simulink model "ATOM_simple_planning_simulator"  (R2026a)
settings: Solver=ode4  StopTime=100  FixedStep=0.01
StopFcn:
  | % Put every new figure in the same MATLAB Figures window as a docked tab.
  | set(groot, 'defaultFigureWindowStyle', 'docked');
  | 
  | if exist('costmap_active', 'var') && ...
  |     exist('vehicle', 'var') && ...
  |     exist('parking_path', 'var') && ...
  |     ~isempty(parking_path)
  | 
  |      plotPlan(costmap_active, vehicle, parking_path);
  | 
  |  else
  | 
  |      warning('No valid parking path is available for plotting.');
  | 
  |  end
  | 
  |  PlotControllerReferences( ...
  |      out.controller_reference_log);
  | 
  |  PlotControllerTracking( ...
  |      out.controller_tracking_log);
  | 
model workspace (MAT data in the model file):
  vehicle : object (value not decoded)
symbols that are objects in the model workspace (value not decoded): vehicle
undefined symbols (not defined in the file): delta_f_LUT, gain4WS_LUT, k_ref_LUT, kappa_gain_BP, Ki, Kp, lateral, longitudinal, planning_validator, rr_gain_BP, rr_LUT, stanley, velocity_smoother
libraries: slpidlib x1
(part 7 of 8)

== matlab function ATOM_simple_planning_simulator/Subsystem2/parkingNMPC ==
  settings: updateMethod=DISCRETE  sampleTime=0.04
  data: tx input; path_length output; ty input; tqz input; tqw input; tdf input; tdr input; tvx input; tax input; max_q output; X input; Y input; s_now output; ey_now output; qz input; qw input; vx input; ax_meas input; df input; dr input; x_now output; veh input; longitudinal_mode output; df_rate_cmd output; dr_rate_cmd output; nmpc_info output; segment_done output; active_segment input; endpoint_error output; a_cmd_history input; costmap input; df_ref_out output; dr_ref_out output; t_ref input; s_ref input; x_ref input; y_ref input; psi_ref input; v_ref input; a_ref input; df_nom input; dr_nom input
function [path_length, max_q, s_now, ey_now, x_now, ...
    longitudinal_mode, df_rate_cmd, dr_rate_cmd, nmpc_info, ...
    segment_done, endpoint_error, ...
    df_ref_out, dr_ref_out] = parkingNMPC( ...
    tx,ty,tqz,tqw,tdf,tdr,tvx,tax, ...
    X,Y,qz,qw,vx,ax_meas,df,dr,veh, ...
    active_segment,a_cmd_history,costmap,t_ref,s_ref,x_ref,y_ref,psi_ref,v_ref,a_ref,df_nom,dr_nom)
%PARKINGNMPC  Steering NMPC of the ATOM parking chain, acados version (row 3).
%
%   Block    : ATOM_parking_chain/Subsystem2/parkingNMPC (MATLAB Function,
%              discrete, sample time Ts = 0.04 s, compiled to C).
%   Role     : computes the FRONT and REAR STEERING-RATE commands of the
%              4WS vehicle. Speed is NOT decided here: the separate block
%              parkingLongitudinalController (feed-forward + P law) computes
%              the acceleration; this block only predicts it.
%   Solver   : the optimal control problem is solved by acados through the
%              Simulink Function 'acadosSolve' (Subsystem2), which wraps
%              the generated S-function acados_solver_sfunction_atom_4ws_nmpc.
%              The OCP itself (model, cost, constraints, solver options) is
%              defined in MATLAB-Autoware/Acados/*.m and generated/compiled
%              by ATOM_Simulink_init.m.
%
%   WHAT HAPPENS EVERY 0.04 s
%     1  Supervisor: reference of the active gear segment, path progress
%        s_now, arrival / stop / wheel-alignment logic, longitudinal mode.
%     2  rolloutForAcados: predict 0.24 s through the steering dead time with
%        the 6 commands already queued (-> initial state x0bar of the OCP),
%        then 1.8 s more with the steering held (-> a_des profile, initial
%        guess, predicted path progress of every node).
%     3  acadosReferences: reference pose/steering of each OCP node, looked
%        up at the predicted path progress (path following).
%     4  buildCorridors: one obstacle-free rectangle per node from the
%        costmap (collision constraints of the OCP).
%     5  callAcados: pack everything into vectors and call acadosSolve
%        (skipped while the wheels are being aligned, status 7).
%     6  Status map: acados status -> controller status; unusable result ->
%        hold steering and stop.
%     7  Apply the FIRST command u0 only (receding horizon) and update the
%        internal copies of the commanded angle and of the delay queue.
%     8  Diagnostics nmpc_info (Scope2 ... Scope7).
%
%   TIMING
%     controller period Ts             0.04 s  (P.controlTs)
%     steering dead time (plant)       0.24 s  = nd = 6 controller steps
%     acceleration dead time (plant)   0.10 s  (handled inside predictStep)
%     OCP: N = 15 intervals of 0.12 s  -> 1.8 s, starting at t + 0.24 s
%
%   INPUTS (29)
%     tx,ty,tqz,tqw,tdf,tdr,tvx,tax  planner trajectory bus fields (x, y,
%                                    qz, qw, front/rear wheel angle, speed,
%                                    acceleration). NOT USED in this version;
%                                    kept so that the block wiring stays the
%                                    same. The reference comes from the
%                                    reference bus (t_ref ... dr_nom).
%     X, Y        [m]     rear-axle centre position (map frame)
%     qz, qw      [-]     yaw quaternion components (psi = 2*atan2(qz,qw))
%     vx          [m/s]   longitudinal speed (rear axle)
%     ax_meas     [m/s^2] longitudinal acceleration
%     df, dr      [rad]   measured front / rear wheel angles
%     veh         [-]     numeric vehicle-parameter vector (vehicleParameters.m)
%     active_segment      index of the gear segment being driven
%     a_cmd_history       3x1 acceleration commands already sent (oldest
%                         first), not yet through the 0.10 s dead time
%     costmap             occupancy-grid bus (info.resolution, width,
%                         height, origin; data int8 H x W: 0 free,
%                         100 occupied, -1 unknown)
%     t_ref, s_ref, x_ref, y_ref, psi_ref, v_ref, a_ref, df_nom, dr_nom
%                         reference of the active segment (time, arc
%                         length, pose, speed, acceleration, nominal
%                         front/rear steering), from the reference bus
%
%   OUTPUTS (13)
%     path_length        length of the active segment [m]       -> Display
%     max_q              max steering variation per metre        -> Display1
%     s_now              path progress [m]       -> longitudinal controller
%     ey_now             lateral error [m] (left +)              -> Scope1
%     x_now              current state [X;Y;psi;vx;df;dr;ax]     -> Display2
%     longitudinal_mode  0 follow plan, 1 slow creep, 2 stop -> long. ctrl
%     df_rate_cmd        front steering-rate command [rad/s]  -> df_cmd out
%     dr_rate_cmd        rear  steering-rate command [rad/s]  -> dr_cmd out
%                        (integrated to an angle by steeringRatetoAngle2,
%                        then delayed 0.24 s before the vehicle model)
%     nmpc_info          6x1 diagnostics (see the end of the main body)
%     segment_done       true when the segment end is reached, stopped and
%                        within the arrival tolerance -> next segment
%     endpoint_error     [distance to segment end [m]; heading error [deg]]
%     df_ref_out, dr_ref_out  reference steering at s_now [rad]
%
%   CONTROLLER STATUS (nmpc_info(6), Scope7)
%     0 acados converged within 0.04 s     1 usable (slow or acados 2)
%     2 unusable -> hold steering, stop    3 baseline mode (use_nmpc false)
%     4 segment done, outside 0.05 m / 2 deg   5 stopped at the end but
%       outside the arrival tolerance 0.20 m / 5 deg
%     7 wheel alignment (vehicle held)     8 cusp hand-off (see note there)
%
%   EXTERNAL DEPENDENCIES
%     acadosSolve     Simulink Function in Subsystem2 (scoped)
%     bicycleGetPose  MATLAB-Autoware/Functions (used by predictStep)

% ---------------------------------------------------------------------
% Persistent state (kept between calls, reset only at simulation start)
%   ref                       reference structure of the active segment
%   s_prev                    path progress of the previous call [m]
%   buf                       6x2 steering-angle commands already sent and
%                             still inside the 0.24 s dead time [front rear],
%                             oldest first
%   terminal_creep_steps      leftover of an earlier version: set but never
%                             read (cleanup candidate)
%   previous_active_segment   to detect a segment change
%   steering_command_state    last commanded angles [front rear] = output
%                             of the external rate-to-angle integrator
%   steering_alignment_pending  true until the wheels reach the start
%                             angles of the new segment
% ---------------------------------------------------------------------
persistent ref s_prev buf terminal_creep_steps
persistent previous_active_segment
persistent steering_command_state
persistent steering_alignment_pending
persistent solver_failure_count

N  = 15;   % OCP intervals; here only the size of U_selected (row 1 is used)
nd = 6;    % steering dead time in controller steps: 0.24 s / 0.04 s

% ===================== 1. SEGMENT BOOKKEEPING =========================
% Detect a change of the active gear segment (forward <-> reverse).
if isempty(previous_active_segment)
    previous_active_segment = active_segment;
    segment_changed = false;
else
    segment_changed = ...
        active_segment ~= previous_active_segment;

    previous_active_segment = active_segment;
end

% Build the reference during the first execution.
if isempty(ref)
    ref = buildRef( ...
        t_ref,s_ref,x_ref,y_ref,psi_ref,v_ref,a_ref, ...
        df_nom,dr_nom);
end

if isempty(s_prev)
    s_prev = 0;
end

if isempty(buf)
    % Initialize the delayed-command history from the measured wheel angles
    % (at start-up nothing different has been commanded yet).
    buf = repmat([df, dr], nd, 1);
end

if isempty(steering_command_state)
    % The commanded angles start equal to the measured wheel angles.
    steering_command_state = [df,dr];
end

% History of acceleration commands already sent to the vehicle.
% Three samples are retained because the acceleration delay is 0.10 s,
% equivalent to 2.5 controller intervals at Ts = 0.04 s.
% Acceleration commands sampled externally every 0.04 seconds.
aBuf = a_cmd_history;

if isempty(terminal_creep_steps)
    terminal_creep_steps = 0.0;
end

if isempty(solver_failure_count)
    solver_failure_count = 0;
end

if isempty(steering_alignment_pending)
    % The first segment also starts with a wheel-alignment check.
    steering_alignment_pending = true;
end

% Rebuild the reference once when the segment changes; restart the path
% progress and request a wheel alignment for the new segment.
if logical(segment_changed)
    ref = buildRef( ...
        t_ref,s_ref,x_ref,y_ref,psi_ref,v_ref,a_ref, ...
        df_nom,dr_nom);
    s_prev = 0;
    terminal_creep_steps = 0.0;
    steering_alignment_pending = true;
end

% ===================== 2. WHERE IS THE CAR ON THE PATH ================
path_length = ref.s(end); max_q = max(ref.q);
[s_new, ey_now] = whereOnPath(ref, X, Y, s_prev);
s_now  = min(max(s_new, s_prev), s_prev + 0.5);   % never backwards, never a big jump forward

% Reference steering at the current progress (outputs for logging).
df_ref_out = lookupS(ref.s, ref.df, s_now);
dr_ref_out = lookupS(ref.s, ref.dr, s_now);

s_prev = s_now;

% --- the state of the car right now ---
psi   = 2*atan2(qz, qw);                              % yaw from the quaternion
x_now = [X; Y; psi; vx; df; dr; ax_meas];             % 7-state vector of the internal prediction model
P     = carNumbers(veh);                              % vehicle, actuator and footprint numbers
M = mapNumbers(costmap);                              % costmap as doubles (0..1, <0 unknown)

% Collision measure of the CURRENT pose (monitor only, Scope2):
% < 0 free, > 0 the expanded footprint overlaps an obstacle cell.
current_collision_constraint = ...
    poseCollisionConstraint(X,Y,psi,P,M);

% Remaining path distance used by the maneuver supervisor.
d_left = max(ref.s(end) - s_now, 0);

% The segment is complete only after reaching its end and stopping.
% Actual distance from the vehicle's rear axle to the segment endpoint.
endpoint_distance = hypot( ...
    X - ref.X(end), ...
    Y - ref.Y(end));

% Heading error relative to the segment endpoint, wrapped to [-pi, pi].
heading_difference = psi - ref.psi(end);

endpoint_heading_error = atan2( ...
    sin(heading_difference), ...
    cos(heading_difference));

% ===================== 3. ARRIVAL, STOP AND ALIGNMENT SUPERVISION =====
%
% Precise tolerance:
% Used to evaluate the final tracking quality.
%
% Arrival tolerance:
% Used to decide whether the stopped vehicle may proceed to the next
% forward/reverse segment.

end_distance_tolerance = 0.05;       % [m]
end_heading_tolerance  = 2*pi/180;   % [rad]

arrive_distance_tolerance = 0.20;    % [m]
arrive_heading_tolerance = 5*pi/180; % [rad]

stop_speed_tolerance = 0.02;         % [m/s]

% Because s_now is not allowed to decrease, end_reached remains true
% after the vehicle reaches the final path progress.
end_reached = ...
    d_left <= 0.02;

% High-accuracy endpoint condition.
pose_acceptable = ...
    (endpoint_distance <= end_distance_tolerance) && ...
    (abs(endpoint_heading_error) <= end_heading_tolerance);

% Practical condition for authorizing the next gear segment.
pose_arrived = ...
    (endpoint_distance <= arrive_distance_tolerance) && ...
    (abs(endpoint_heading_error) <= arrive_heading_tolerance);

% The vehicle must be nearly stationary before changing segments.
stopped = ...
    abs(vx) <= stop_speed_tolerance;

% Steering must be positioned for the new segment before motion begins.
steering_alignment_tolerance = 2*pi/180;

segment_start_front_steering = ref.df(1);
segment_start_rear_steering  = ref.dr(1);

front_steering_aligned = ...
    abs(df-segment_start_front_steering) <= ...
    steering_alignment_tolerance;

rear_steering_aligned = ...
    abs(dr-segment_start_rear_steering) <= ...
    steering_alignment_tolerance;

steering_aligned = ...
    front_steering_aligned && ...
    rear_steering_aligned;

% Release the alignment hold only after the measured wheels - not merely
% the requested commands - have reached the new segment's starting angles.
if steering_alignment_pending && stopped && steering_aligned
    steering_alignment_pending = false;
end

steering_alignment_active = steering_alignment_pending;

% Advance to the next segment only after reaching the endpoint progress,
% stopping, and satisfying the practical arrival tolerance.
segment_done = ...
    end_reached && ...
    stopped && ...
    pose_arrived;

% If the vehicle stops outside the arrival tolerance, keep the current
% segment active and report the failure through the controller status.
arrival_failed = ...
    end_reached && ...
    stopped && ...
    ~pose_arrived;

% Permanent endpoint diagnostics:
%   element 1: position error [m]
%   element 2: signed heading error [deg]
endpoint_error = [ ...
    endpoint_distance; ...
    endpoint_heading_error*180/pi];

% Longitudinal modes (read by parkingLongitudinalController):
%   0 = follow the planned velocity profile
%   1 = slow terminal approach
%   2 = stop
longitudinal_mode = 0.0;

if steering_alignment_active

    % Keep the vehicle stopped while the wheels align.
    longitudinal_mode = 2.0;

elseif end_reached

    if pose_arrived
        % Correct endpoint pose reached.
        longitudinal_mode = 2.0;
    else
        % Continue slowly to correct the endpoint pose.
        % S1: creep only while the endpoint is still ahead in the driving
        % direction, and for at most max_creep_steps samples
        % (150 x 0.04 s = 6 s, i.e. 0.30 m at 0.05 m/s). Otherwise stop;
        % once stopped, arrival_failed reports controller status 5.
        max_creep_steps = 150;
        endpoint_ahead = ref.gear*( ...
            cos(psi)*(ref.X(end) - X) + sin(psi)*(ref.Y(end) - Y));
        if endpoint_ahead <= 0.02
            % Endpoint beside or behind the car: creeping cannot reach it.
            terminal_creep_steps = max_creep_steps;
        end
        if terminal_creep_steps < max_creep_steps
            terminal_creep_steps = terminal_creep_steps + 1;
            longitudinal_mode = 1.0;
        else
            % Creep abandoned: stop (latched until the segment changes).
            longitudinal_mode = 2.0;
        end
    end

end

% ===================== 4. STEERING: acados NMPC =======================
use_nmpc = true;      % false = D1 baseline (follow the plan blindly)

if use_nmpc

    % Collision tolerance of the cusp hand-off check (section 4.6).
    collision_tolerance = 1e-6;

    % ---- 4.1 Prediction that prepares the OCP -----------------------
    % Phase 1: 0.24 s with the 6 queued commands -> x0bar (OCP state at
    % t + 0.24 s). Phase 2: 15 x 0.12 s with the steering held ->
    % aDes (acceleration entering the lag, per interval), xGuess
    % (initial guess) and sNode (predicted path progress of each node).
    [x0bar, aDes, xGuess, sNode] = rolloutForAcados( ...
        x_now, aBuf, buf, steering_command_state, ...
        s_now, ref, P, longitudinal_mode);

    % ---- 4.2 References at the predicted path progress of each node --
    acados_reference = acadosReferences(ref, sNode);

    % ---- 4.3 Obstacle corridor for every node, from the costmap -------
    [Acorr, bcorr] = buildCorridors(x0bar, acados_reference, P, M);

    % ---- 4.4 Solve with acados ----------------------------------------
    % Skipped while the supervisor aligns the wheels (status 7): the
    % steering command is overridden by the alignment logic anyway.
    if steering_alignment_active
        u0_acados       = zeros(2,1);
        acados_status   = 0;
        acados_sqp_iter = 0;
        solve_time      = 0;
    else
        [u0_acados, ~, acados_status, acados_sqp_iter, solve_time] = ...
            callAcados(x0bar, acados_reference, aDes, xGuess, Acorr, bcorr);
    end

    % ---- 4.5 Check the returned first command and map the status ------
    acados_rate_bound = 1.0;    % must equal atomCfg.omegaMax (compiled in the solver)
    finite_solution = all(isfinite(u0_acados));
    inside_bounds   = all(abs(u0_acados) <= acados_rate_bound + 1e-6);

    % Translate the acados status into the controller status.
    %   acados 0           -> 0 (1 if slower than the 0.04 s period)
    %   acados 2 (max it.) -> 1 (usable, not fully converged)
    %   anything else      -> 2 (unusable)
    if acados_status == 0 && finite_solution && inside_bounds
        if solve_time > P.controlTs
            controller_status = 1;
        else
            controller_status = 0;
        end
    elseif acados_status == 2 && finite_solution && inside_bounds
        controller_status = 1;
    else
        controller_status = 2;
    end

    % Endpoint-arrival diagnostics (same as the fmincon version).
    % S3: a non-converged solve (acados status ~= 0) is accepted only
    % for a short time. After more than max_solver_failures consecutive
    % failures (5 x 0.04 s = 0.2 s) the command is treated as unusable:
    % controller status 2 -> hold the steering and stop. The stop is
    % latched: once triggered, the counter is no longer reset.
    max_solver_failures = 5;
    if solver_failure_count <= max_solver_failures
        if acados_status ~= 0
            solver_failure_count = solver_failure_count + 1;
        else
            solver_failure_count = 0;
        end
    end
    if solver_failure_count > max_solver_failures
        controller_status = 2;
    end

    % Endpoint-arrival diagnostics (same as the fmincon version).
    if controller_status ~= 2
        if arrival_failed
            controller_status = 5;
        elseif segment_done && ~pose_acceptable
            controller_status = 4;
        end
    end

    % Steering-rate plan used by the rest of the function. Only the FIRST
    % row is applied (receding horizon); the other rows stay zero.
    % Status 2: rate 0 = hold the last issued steering command.
    U_selected = zeros(N,2);
    if controller_status ~= 2
        U_selected(1,1:2) = u0_acados(:).';
    else
        % No valid (collision-free) steering plan: hold steering and stop.
        longitudinal_mode = 2.0;
    end

    % ---- Wheel alignment at a gear change (status 7) ------------------
    % Align the wheels directly while the vehicle is stopped. This does not
    % move the vehicle body. While steering alignment is pending, keep the
    % vehicle stopped and do not allow the NMPC solution to compete with it.
    if steering_alignment_active

        longitudinal_mode = 2.0;
        controller_status = 7;

        % Zero rate holds the current desired steering angles while the
        % vehicle is still coming to rest.
        U_selected = zeros(N,2);

        % Begin changing the steering only after the vehicle has stopped:
        % rate that reaches the start angles in one step, limited to the
        % actuator rate limit P.rateLim (5 rad/s).
        if stopped

            target_front_angle = max( ...
                -P.steerMax, ...
                min(P.steerMax,segment_start_front_steering));

            target_rear_angle = max( ...
                -P.steerMax, ...
                min(P.steerMax,segment_start_rear_steering));

            alignment_front_rate = ...
                (target_front_angle-steering_command_state(1))/P.controlTs;

            alignment_rear_rate = ...
                (target_rear_angle-steering_command_state(2))/P.controlTs;

            alignment_front_rate = max( ...
                -P.rateLim, ...
                min(P.rateLim,alignment_front_rate));

            alignment_rear_rate = max( ...
                -P.rateLim, ...
                min(P.rateLim,alignment_rear_rate));

            U_selected(1,1:2) = ...
                [alignment_front_rate,alignment_rear_rate];
        end
    end

    % ---- Outputs: the two steering-rate commands -----------------------
    selected_input = U_selected(1,:);

    df_rate_cmd = selected_input(1);
    dr_rate_cmd = selected_input(2);

    selected_rate = selected_input(1:2);

    % Mirror the external rate-to-angle integrator (steeringRatetoAngle2)
    % inside the NMPC: commanded angle after this step.
    sent_angle_trajectory = expandSteeringRatePlan( ...
        selected_rate,steering_command_state,P);

    steering_command_state = ...
        sent_angle_trajectory(end,:);

    % Push the new command into the 0.24 s delay queue (keep the last 6).
    updated_delay_history = ...
        [buf;sent_angle_trajectory];

    buf = updated_delay_history(end-nd+1:end,:);

    % Status 7 means the vehicle is intentionally stationary while its
    % measured steering aligns with the new segment.
    if steering_alignment_active && ...
            (controller_status == 0 || controller_status == 1)

        controller_status = 7;
    end

    % ---- 4.6 Cusp hand-off (status 8) ---------------------------------
    % Terminal creep is collision-infeasible, but the stopped vehicle is
    % currently collision-free and sufficiently close to the cusp.
    % Authorize the gear change so the next segment can move away from
    % the obstacle instead of repeating an impossible creep forever.
    % NOTE: this needs controller_status == 6, which only the fmincon
    % version produced. In this acados version it can never trigger.

    cusp_recovery_distance_tolerance = 0.25;        % [m]
    cusp_recovery_heading_tolerance  = 10*pi/180;   % [rad]

    safe_cusp_handoff = ...
        (controller_status == 6) && ...
        arrival_failed && ...
        ~steering_alignment_active && ...
        (current_collision_constraint <= collision_tolerance) && ...
        (endpoint_distance <= cusp_recovery_distance_tolerance) && ...
        (abs(endpoint_heading_error) <= ...
        cusp_recovery_heading_tolerance);

    if safe_cusp_handoff
        segment_done = true;
        controller_status = 8;
    end

    % ---- 4.7 Diagnostics (Demux -> Scope2 ... Scope7) -----------------
    %   1 collision monitor of the CURRENT pose (> 0 = overlaps an obstacle)
    %   2 acados status (0 converged, 2 max iterations, 4 QP failure, ...)
    %   3 acados CPU time [s]
    %   4 SQP iterations
    %   5 acceleration entering the lag at node 0 (a_des) [m/s^2]
    %   6 controller status
    nmpc_info = [ ...
        double(current_collision_constraint); ...
        double(acados_status); ...
        double(solve_time); ...
        double(acados_sqp_iter); ...
        double(aDes(1)); ...
        double(controller_status)];
else
    % ===================== BASELINE (use_nmpc = false) ===================
    % Follow the planned steering angles at the current progress, without
    % optimisation (comparison mode only).
    target_front_angle = lookupS(ref.s,ref.df,s_now);
    target_rear_angle  = lookupS(ref.s,ref.dr,s_now);

    % Convert the required angle changes into steering-rate commands.
    df_rate_cmd = ...
        (target_front_angle-steering_command_state(1))/P.controlTs;

    dr_rate_cmd = ...
        (target_rear_angle-steering_command_state(2))/P.controlTs;

    % Apply the actuator steering-rate limit.
    df_rate_cmd = max(-P.rateLim,min(P.rateLim,df_rate_cmd));
    dr_rate_cmd = max(-P.rateLim,min(P.rateLim,dr_rate_cmd));

    % Mirror the steering command actually selected in baseline mode.
    selected_rate = [df_rate_cmd,dr_rate_cmd];

    sent_angle_trajectory = expandSteeringRatePlan( ...
        selected_rate,steering_command_state,P);

    steering_command_state = sent_angle_trajectory(end,:);

    updated_delay_history = [buf;sent_angle_trajectory];
    buf = updated_delay_history(end-nd+1:end,:);

    nmpc_info = [0; 0; 0; 0; 0; 3];
end
end

%==========================================================================
%  GENERAL HELPERS (vehicle numbers, costmap, prediction model, path)
%==========================================================================

%--------------------------------------------------------------------------
function P = carNumbers(veh)
%CARNUMBERS  Vehicle, actuator, timing and footprint numbers in one struct.
%   veh is the numeric vector of vehicleParameters.m:
%     veh(3) wheel base, veh(4) track, veh(5)/veh(6) front/rear overhang,
%     veh(7)/veh(8) left/right overhang, veh(10) max wheel angle,
%     veh(15) velocity limit, veh(16) acceleration limit,
%     veh(18) actuator steering-rate limit, veh(19) acceleration dead time,
%     veh(20) acceleration time constant, veh(22) steering time constant.
%   All fields must be created before the structure is read (code generation).

collisionMargin = 0.4;%0.5;     % total margin around the car [m] (0.25 m per face)

% Controller and internal prediction timing.
controlTs    = 0.04;
predictionTs = 0.04;

P.L        = veh(3);       % wheel base 2.0 m
P.steerMax = veh(10);      % max wheel / command angle 0.70 rad
P.aMax     = veh(16);      % acceleration clip in the prediction 7.0 m/s^2
P.rateLim  = veh(18);      % actuator steering-rate limit 5 rad/s
P.tau      = veh(22);      % steering time constant 0.27 s

% Speed clip of the prediction. veh(15) is the simulator velocity limit
% (50 m/s), so in practice this clip is never active.
P.vMax = veh(15);       % Prediction clip
P.vStateMax = veh(15);  % leftover of the fmincon speed constraint: not used any more

P.controlTs = controlTs;
P.predictionTs = predictionTs;
P.substepsPerControl = round( ...
    controlTs/predictionTs);   % = 1: one prediction step per command

P.accDelay = veh(19);      % 0.10 s; not used: the delay is built into predictStep / aBuf
P.accTau   = veh(20);      % acceleration time constant 0.10 s
P.aCmdMax  = 1.0; % Match a_cmd_limit in parkingLongitudinalController.

% Expanded footprint in vehicle coordinates (origin = rear-axle centre,
% l forward, w to the left): l in [footprintBack, footprintFront],
% w in [-footprintHalfWidth, +footprintHalfWidth].
P.footprintMargin = collisionMargin;     % not used elsewhere

P.footprintBack = ...
    -(veh(6) + collisionMargin/2);         % -0.71 m

P.footprintFront = ...
    veh(3) + veh(5) + collisionMargin/2;   % +2.71 m

P.footprintHalfWidth = ...
    (veh(4) + veh(7) + veh(8) + collisionMargin)/2;   % 1.328 m
end

%--------------------------------------------------------------------------
function M = mapNumbers(costmap)
%MAPNUMBERS  Costmap bus -> doubles used by the collision code.
%   Cell (ix, iy), zero-based, is a square of side res centred at
%   (originX + ix*res, originY + iy*res). grid = data/100:
%   0 free, 1 occupied, -0.01 unknown (unknown is treated as an obstacle).

resolution = double(costmap.info.resolution);

M.res = resolution;
M.width = double(costmap.info.width);
M.height = double(costmap.info.height);

M.originX = double(costmap.info.origin.position.x);
M.originY = double(costmap.info.origin.position.y);

M.grid = double(costmap.data)/100;

M.cellHalf = resolution/2;
end

%--------------------------------------------------------------------------
function [x1,aBuf1,df_raw,dr_raw,vx_raw] = predictStep( ...
    x0,aBuf,aCmd,dfc,drc,P)
%PREDICTSTEP  Discrete vehicle model over one 0.04 s controller interval.
%   x0   = [X; Y; psi; vx; df; dr; ax]   state at the start of the step
%   aBuf = acceleration commands inside the 0.10 s dead time (oldest first)
%   aCmd = acceleration command issued in this step (enters aBuf)
%   dfc, drc = steering-angle commands reaching the actuator in this step
%   x1   = state after 0.04 s;  aBuf1 = updated acceleration queue.
%   df_raw, dr_raw, vx_raw are the unclipped values (were used by the
%   fmincon constraints; the acados roll-out does not use them).
%   This is the model used to compute x0bar, a_des and the initial guess.

X   = x0(1);
Y   = x0(2);
psi = x0(3);
vx  = x0(4);
df  = x0(5);
dr  = x0(6);
ax  = x0(7);

%% Steering actuator: first-order lag (tau = 0.27 s) with rate limit
ddf = max( ...
    -P.rateLim, ...
    min(P.rateLim,(dfc-df)/P.tau));

ddr = max( ...
    -P.rateLim, ...
    min(P.rateLim,(drc-dr)/P.tau));

df_raw = df + P.predictionTs*ddf;
dr_raw = dr + P.predictionTs*ddr;

df1 = max(-P.steerMax,min(P.steerMax,df_raw));
dr1 = max(-P.steerMax,min(P.steerMax,dr_raw));

%% Acceleration delay and actuator lag

% The 0.04 s interval is divided into two 0.02 s parts.
h = 0.5*P.predictionTs;

% For a 0.10 s transport delay, the delayed command changes halfway
% through the current 0.04 s interval.
aDelayedFirst  = aBuf(1);
aDelayedSecond = aBuf(2);

% First half of the acceleration-actuator response.
axHalf = ax + ...
    h*(aDelayedFirst-ax)/P.accTau;

axHalf = max( ...
    -P.aMax, ...
    min(P.aMax,axHalf));

% Second half of the acceleration-actuator response.
ax1 = axHalf + ...
    h*(aDelayedSecond-axHalf)/P.accTau;

ax1 = max( ...
    -P.aMax, ...
    min(P.aMax,ax1));

% Integrate longitudinal acceleration over the two half-steps (trapezoid).
deltaVFirst = ...
    0.5*h*(ax+axHalf);

deltaVSecond = ...
    0.5*h*(axHalf+ax1);

vxFromAcceleration = ...
    vx + deltaVFirst + deltaVSecond;

% Steering changes during this controller interval, so use its
% midpoint value when predicting the vehicle motion.
dfMid = 0.5*(df+df1);
drMid = 0.5*(dr+dr1);

% Match the longitudinal-velocity equation used by Vehicle_Model:
% dvx/dt = a + yawRate * v * sin(dr), with v = vx / cos(dr).
vxMidForCoupling = ...
    0.5*(vx+vxFromAcceleration);

vehicleSpeedMid = ...
    vxMidForCoupling/max(cos(drMid),0.1);

yawRateMid = ...
    (vxMidForCoupling/P.L) * ...
    (tan(dfMid)-tan(drMid));

rearSteeringVelocityTerm = ...
    yawRateMid*vehicleSpeedMid*sin(drMid);

% Unclipped prediction (returned as vx_raw).
vx_raw = vxFromAcceleration + ...
    P.predictionTs*rearSteeringVelocityTerm;

% Keep the numerical guard for state propagation.
vx1 = max(-P.vMax,min(P.vMax,vx_raw));

% Store the acceleration command predicted for the current cycle.
aBuf1 = [aBuf(2:end); aCmd];

%% Vehicle motion: arc of the rear-axle point (bicycleGetPose)

vxMid = 0.5*(vx+vx1);

dRear = ...
    vxMid*P.predictionTs/max(cos(drMid),0.1);   % distance travelled by the rear-axle point

[X1,Y1,psi1] = bicycleGetPose( ...
    X,Y,psi,dfMid,drMid,P.L,dRear);


x1 = [X1;Y1;psi1;vx1;df1;dr1;ax1];


end

%-------------------------------------------------------------------------
function angle_commands = expandSteeringRatePlan( ...
    rate_commands,initial_angle_command,P)
%EXPANDSTEERINGRATEPLAN  Integrate steering-rate commands into angles.
%   Same law as the external block steeringRatetoAngle2:
%     c(k+1) = sat( c(k) + 0.04 * sat(rate, +-P.rateLim), +-P.steerMax )
%   rate_commands: n x 2 [front rear] rates; initial_angle_command: 1 x 2.
%   angle_commands: (n*substeps) x 2 commanded angles after each sub-step.
%   Called with one row (the command applied now): the result updates
%   steering_command_state and the delay queue buf.

number_of_rate_commands = size(rate_commands,1);
substeps_per_command = P.substepsPerControl;

number_of_angle_samples = ...
    number_of_rate_commands*substeps_per_command;

angle_commands = zeros(number_of_angle_samples,2);

front_command = initial_angle_command(1);
rear_command  = initial_angle_command(2);

sample_index = 0;

for k = 1:number_of_rate_commands

    front_rate = max( ...
        -P.rateLim, ...
        min(P.rateLim,rate_commands(k,1)));

    rear_rate = max( ...
        -P.rateLim, ...
        min(P.rateLim,rate_commands(k,2)));

    for j = 1:substeps_per_command

        front_command = max( ...
            -P.steerMax, ...
            min(P.steerMax, ...
            front_command + ...
            P.predictionTs*front_rate));

        rear_command = max( ...
            -P.steerMax, ...
            min(P.steerMax, ...
            rear_command + ...
            P.predictionTs*rear_rate));

        sample_index = sample_index + 1;

        angle_commands(sample_index,1) = front_command;
        angle_commands(sample_index,2) = rear_command;
    end
end
end

%--------------------------------------------------------------------------
function a_cmd = longitudinalCommandPrediction( ...
    ref, s, vx, longitudinal_mode, P)
%LONGITUDINALCOMMANDPREDICTION  Copy of the law of parkingLongitudinalController.
%   Predicts the acceleration command the separate longitudinal controller
%   will issue at progress s and speed vx:
%     a_cmd = sat( a_ff + Kp*(v_ref - vx), +-P.aCmdMax )
%   mode 0: plan (v_ref, a_ref at s, Kp = 1); mode 1: creep at 0.05 m/s in
%   the segment gear; mode 2: stop (v_ref = 0, Kp_stop = 5).
%   Braking feed-forward is dropped while the car is already slower than
%   its reference in the gear direction.

Kp = 1.0;
Kp_stop = 5.0;
terminal_creep_speed = 0.05;

v_ref = lookupS(ref.s,ref.v,s);
a_ref = lookupS(ref.s,ref.a,s);

gear = ref.gear;             % +1 forward, -1 reverse
Kp_active = Kp;

if longitudinal_mode == 2.0

    % Stop mode.
    v_ref = 0.0;
    a_ref = 0.0;
    Kp_active = Kp_stop;

elseif longitudinal_mode == 1.0

    % Terminal-creep mode.
    v_ref = gear*terminal_creep_speed;
    a_ref = 0.0;

end

speed_error = v_ref-vx;

speed_in_gear = gear*vx;
reference_speed_in_gear = gear*v_ref;
feedforward_in_gear = gear*a_ref;

a_feedforward = a_ref;

% Apply braking feedforward only while the vehicle is moving faster
% than its reference in the intended gear direction.
if feedforward_in_gear < 0.0 && ...
        speed_in_gear <= reference_speed_in_gear

    a_feedforward = 0.0;

end

a_unsaturated = ...
    a_feedforward + Kp_active*speed_error;

a_cmd = max( ...
    -P.aCmdMax, ...
    min(P.aCmdMax,a_unsaturated));

end

%--------------------------------------------------------------------------
function v = lookupS(sv, vv, s)
%LOOKUPS  Linear interpolation of vv(sv) at s, held constant outside the range.
%   Used for every reference lookup by arc length (or by time).
n = numel(sv);
v = vv(n);
if s <= sv(1), v = vv(1); return; end
if s >= sv(n), return; end
for i = 1:n-1
    if s <= sv(i+1)
        ds = sv(i+1) - sv(i);
        if ds < 1e-12
            v = vv(i+1);
        else
            v = vv(i) + (s - sv(i))/ds*(vv(i+1) - vv(i));
        end
        return;
    end
end
end

%--------------------------------------------------------------------------
function ref = buildRef( ...
    t_ref,s_ref,x_ref,y_ref,psi_ref,v_ref,a_ref, ...
    df_nom,dr_nom)
%BUILDREF  Reference structure of the active segment.
%   Fields: t, s, X, Y, psi, v, a, df, dr (column vectors), q = steering
%   variation per metre (max over front/rear), gear = sign of the first
%   non-zero reference speed (+1 forward, -1 reverse).

% Local arrays
t   = t_ref(:);
s   = s_ref(:);
Xr  = x_ref(:);
Yr  = y_ref(:);
psir = psi_ref(:);
vr  = v_ref(:);
ar  = a_ref(:);
dfr = df_nom(:);
drr = dr_nom(:);

n = numel(t);

%% Steering variation per metre

q = zeros(n,1);

for i = 1:n-1

    ds = max(s(i+1)-s(i),1e-9);

    q(i) = max( ...
        abs(dfr(i+1)-dfr(i)), ...
        abs(drr(i+1)-drr(i))) / ds;

end

if n > 1
    q(n) = q(n-1);
else
    q(1) = 0.0;
end

%% Forward or reverse gear

gear = 1;

for i = 1:n

    if abs(vr(i)) > 1e-6
        gear = sign(vr(i));
        break;
    end

end

%% Create every structure field after calculations are complete

ref.t    = t;
ref.s    = s;
ref.X    = Xr;
ref.Y    = Yr;
ref.psi  = psir;
ref.v    = vr;
ref.a    = ar;
ref.df   = dfr;
ref.dr   = drr;
ref.q    = q;
ref.gear = gear;

end

%--------------------------------------------------------------------------
function [s, ey] = whereOnPath(ref, X, Y, s_guess)
%WHEREONPATH  Closest point on the route to (X,Y).
%   s  : how far along the route that point is [m]
%   ey : how far to the side the car is (left positive) [m]
%   First searches the segments within 1.5 m of s_guess; if none is found,
%   searches the whole route.
n = numel(ref.s);
best = inf;  s = s_guess;  ey = 0;
win  = 1.5;

for pass = 1:2
    for i = 1:n-1
        if abs(ref.s(i) - s_guess) > win
            continue;
        end
        ax = ref.X(i);   ay = ref.Y(i);
        bx = ref.X(i+1); by = ref.Y(i+1);
        L2 = (bx-ax)^2 + (by-ay)^2;
        t  = ((X-ax)*(bx-ax) + (Y-ay)*(by-ay)) / max(L2, 1e-12);
        t  = min(max(t, 0), 1);
        px = ax + t*(bx-ax);   py = ay + t*(by-ay);
        d2 = (X-px)^2 + (Y-py)^2;
        if d2 < best
            best = d2;
            s  = ref.s(i) + t*(ref.s(i+1) - ref.s(i));
            ey = sign((bx-ax)*(Y-ay) - (by-ay)*(X-ax)) * sqrt(d2);
        end
    end
    if best < inf, break; end
    win = inf;
end
end

%--------------------------------------------------------------------------
function cPose = poseCollisionConstraint(X,Y,psi,P,M)
%POSECOLLISIONCONSTRAINT  Collision measure of ONE vehicle pose (SAT test).
%   In this version it is only a MONITOR of the current pose (Scope2 and the
%   cusp check); the OCP uses the corridors of buildCorridors instead.
%     cPose < 0 : collision-free (about minus the clearance, >= -1 m)
%     cPose = 0 : touching an obstacle cell or the map boundary
%     cPose > 0 : the expanded footprint overlaps an obstacle / leaves the map
%   Separating-axis test between the expanded footprint rectangle and every
%   occupied or unknown cell near the car (world axes and vehicle axes).

% Nearby obstacles begin influencing the constraint from this distance.
% This is not an additional vehicle safety margin.
influenceDistance = 1.0;

% Prevent exact geometric touching from being accepted because of
% numerical round-off.
numericalClearance = 1e-4;

ct = cos(psi);
st = sin(psi);

%% Enlarged vehicle rectangle

back = P.footprintBack;
front = P.footprintFront;
halfWidth = P.footprintHalfWidth;

vehicleCentreOffset = 0.5*(front + back);
vehicleHalfLength = 0.5*(front - back);

vehicleCentreX = X + ct*vehicleCentreOffset;
vehicleCentreY = Y + st*vehicleCentreOffset;

% Projection of the rotated vehicle rectangle onto the world axes.
vehicleProjectionX = ...
    vehicleHalfLength*abs(ct) + halfWidth*abs(st);

vehicleProjectionY = ...
    vehicleHalfLength*abs(st) + halfWidth*abs(ct);

vehicleMinX = vehicleCentreX - vehicleProjectionX;
vehicleMaxX = vehicleCentreX + vehicleProjectionX;
vehicleMinY = vehicleCentreY - vehicleProjectionY;
vehicleMaxY = vehicleCentreY + vehicleProjectionY;

%% Map-boundary constraint

mapMinX = M.originX - M.cellHalf;
mapMaxX = M.originX + (M.width-1)*M.res + M.cellHalf;

mapMinY = M.originY - M.cellHalf;
mapMaxY = M.originY + (M.height-1)*M.res + M.cellHalf;

boundaryConstraint = max( ...
    max( ...
        mapMinX - vehicleMinX, ...
        vehicleMaxX - mapMaxX), ...
    max( ...
        mapMinY - vehicleMinY, ...
        vehicleMaxY - mapMaxY));

%% Find nearby costmap cells

searchHalfX = ...
    vehicleProjectionX + M.cellHalf + influenceDistance;

searchHalfY = ...
    vehicleProjectionY + M.cellHalf + influenceDistance;

ix0 = ceil( ...
    (vehicleCentreX-searchHalfX-M.originX)/M.res);

ix1 = floor( ...
    (vehicleCentreX+searchHalfX-M.originX)/M.res);

iy0 = ceil( ...
    (vehicleCentreY-searchHalfY-M.originY)/M.res);

iy1 = floor( ...
    (vehicleCentreY+searchHalfY-M.originY)/M.res);

ix0 = max(0,ix0);
ix1 = min(M.width-1,ix1);

iy0 = max(0,iy0);
iy1 = min(M.height-1,iy1);

% A value of -influenceDistance is safely feasible.
obstacleConstraint = -influenceDistance;

% Projection of a square costmap cell onto either vehicle axis.
cellProjectionRotated = ...
    M.cellHalf*(abs(ct) + abs(st));

%% Rectangle-versus-cell constraints

if ix0 <= ix1 && iy0 <= iy1

    for iy = iy0:iy1
        for ix = ix0:ix1

            cellValue = M.grid(iy+1,ix+1);

            % Occupied cells are >= 1.
            % Unknown cells are negative and are also unsafe.
            if cellValue >= 1.0 || cellValue < 0.0

                cellX = M.originX + ix*M.res;
                cellY = M.originY + iy*M.res;

                dx = cellX - vehicleCentreX;
                dy = cellY - vehicleCentreY;

                % Overlap on the two world axes.
                overlapWorldX = ...
                    vehicleProjectionX + M.cellHalf - abs(dx);

                overlapWorldY = ...
                    vehicleProjectionY + M.cellHalf - abs(dy);

                % Cell position expressed along the vehicle axes.
                distanceLongitudinal = ct*dx + st*dy;
                distanceLateral = -st*dx + ct*dy;

                % Overlap on the two vehicle axes.
                overlapLongitudinal = ...
                    vehicleHalfLength + ...
                    cellProjectionRotated - ...
                    abs(distanceLongitudinal);

                overlapLateral = ...
                    halfWidth + ...
                    cellProjectionRotated - ...
                    abs(distanceLateral);

                % SAT collision measure for this occupied cell:
                % the smallest overlap over the four axes (negative = gap).
                cellConstraint = min( ...
                    min(overlapWorldX,overlapWorldY), ...
                    min(overlapLongitudinal,overlapLateral));

                obstacleConstraint = max( ...
                    obstacleConstraint, ...
                    cellConstraint);
            end
        end
    end
end

% The worst condition determines whether this pose is feasible.
cPose = ...
    max(boundaryConstraint,obstacleConstraint) + ...
    numericalClearance;
end

%==========================================================================
%  acados HELPERS (prepare the OCP data, call the solver, build corridors)
%
%  OCP solved by acados (defined in MATLAB-Autoware/Acados):
%    state  x = [X Y psi vx df dr a cF cR]  (cF, cR = commanded angles)
%    input  u = [d(cF)/dt  d(cR)/dt]        (bounds +-1 rad/s)
%    param  p = [a_des; A(:); b; eps]       (17 per node)
%    N = 15 intervals of 0.12 s, node k at time t + 0.24 + 0.12*k
%    cost: weighted tracking of [X Y psi df dr] + small rate penalty,
%    soft corridor constraints A*corner - b <= 0 for the 4 corners.
%  MATLAB column k (k = 1..16) of every per-node array = acados node k-1.
%==========================================================================

%--------------------------------------------------------------------------
function [x1, aBuf1, s1, mode1] = rolloutStep( ...
    x, aBuf, s, mode0, dfc, drc, ref, P)
%ROLLOUTSTEP  One 0.04 s step of the closed-loop prediction.
%   Stop-mode check -> predicted longitudinal command -> vehicle model
%   (predictStep) -> new path progress (whereOnPath).
%   x = [X;Y;psi;vx;df;dr;ax], dfc/drc = steering commands reaching the
%   actuator in this step, mode0 = longitudinal mode at the start.

mode1 = mode0;

% Within 2 cm of the segment end the longitudinal controller stops the car
% (unless it is in creep mode 1).
if max(ref.s(end)-s, 0.0) <= 0.02 && mode1 ~= 1.0
    mode1 = 2.0;
end

aCmd = longitudinalCommandPrediction(ref, s, x(4), mode1, P);

[x1, aBuf1] = predictStep(x, aBuf, aCmd, dfc, drc, P);

[s1, ~] = whereOnPath(ref, x1(1), x1(2), s);
end

%--------------------------------------------------------------------------
function [x0bar, aDes, xGuess, sNode] = rolloutForAcados( ...
    x_now, aBuf, buf, steering_command_state, s_now, ref, P, longitudinal_mode)
%ROLLOUTFORACADOS  Forward simulation that prepares the acados problem.
%
% Phase 1, 0 ... 0.24 s (delay compensation):
%   the 6 steering commands already inside the dead time (buf, oldest
%   first) reach the wheels whatever we decide now -> predicted state at
%   t + 0.24 s. The OCP starts there:
%     x0bar = [ x(t+0.24) ; last issued commanded angles ]   (9 x 1)
% Phase 2, 0.24 ... 2.04 s (15 acados intervals of 0.12 s = 3 steps each):
%   steering command held at the last issued value; the longitudinal loop
%   is predicted with the same law as the real controller ->
%     aDes(k)  : mean acceleration command entering the lag in interval k
%                (parameter p(1) of node k-1)
%     xGuess   : 9 x 16 initial guess of the OCP states
%     sNode(k) : predicted path progress of node k-1 (sNode(1) at x0bar)

nd       = 6;      % 0.24 s / 0.04 s
Nac      = 15;     % acados intervals
nPerNode = 3;      % 0.12 s / 0.04 s

x     = x_now;     % [X; Y; psi; vx; df; dr; a]
s     = s_now;
aBufP = aBuf;
modeP = longitudinal_mode;

cmdHeld = steering_command_state(:);   % last issued steering command [front; rear]

% ---- Phase 1: through the steering dead time ----
for j = 1:nd
    [x, aBufP, s, modeP] = rolloutStep( ...
        x, aBufP, s, modeP, buf(j,1), buf(j,2), ref, P);
end

x0bar = [x; cmdHeld];                  % acados initial state (9 x 1)
sNode    = zeros(1, Nac+1);            % predicted path progress at each node
sNode(1) = s;

% ---- Phase 2: over the acados horizon ----
aDes   = zeros(1, Nac+1);
xGuess = zeros(9, Nac+1);
xGuess(:,1) = x0bar;

for k = 1:Nac
    aSum = 0.0;
    for j = 1:nPerNode
        % predictStep feeds aBuf(1), then aBuf(2) to the lag (0.02 s each)
        aSum = aSum + 0.5*(aBufP(1) + aBufP(2));
        [x, aBufP, s, modeP] = rolloutStep( ...
            x, aBufP, s, modeP, cmdHeld(1), cmdHeld(2), ref, P);
    end
    aDes(k)       = aSum/nPerNode;      % mean over the 0.12 s interval
    xGuess(:,k+1) = [x; cmdHeld];
    sNode(k+1)    = s;
end

aDes(Nac+1) = aDes(Nac);               % terminal node: no dynamics, not used
end

%--------------------------------------------------------------------------
function reference = acadosReferences(ref, sNode)
%ACADOSREFERENCES  Reference of every OCP node, by PATH PROGRESS.
%   reference(:,k) = [X; Y; psi; deltaF; deltaR] of the reference at the
%   predicted progress sNode(k) (column k = acados node k-1).
%   Path-following form: the reference point is where the car is predicted
%   to be along the path, so the steering only has to remove lateral and
%   heading errors; timing (along-path) errors belong to the longitudinal
%   controller. psi is unwrapped so that interpolation never jumps at +-pi.

Nac = 15;

psiUnwrapped = unwrap(ref.psi);        % no jump at +-pi when interpolating

reference = zeros(5, Nac+1);

for k = 1:Nac+1
    sk = min(max(sNode(k), ref.s(1)), ref.s(end));   % stay inside the segment

    reference(1,k) = lookupS(ref.s, ref.X,        sk);
    reference(2,k) = lookupS(ref.s, ref.Y,        sk);
    reference(3,k) = lookupS(ref.s, psiUnwrapped, sk);
    reference(4,k) = lookupS(ref.s, ref.df,       sk);
    reference(5,k) = lookupS(ref.s, ref.dr,       sk);
end
end

%--------------------------------------------------------------------------
function [u0, Uopt, solverStatus, sqpIter, solveTime] = callAcados( ...
    x0bar, reference, aDes, xGuess, Acorr, bcorr)
%CALLACADOS  Pack the OCP data and solve it with the acados S-function.
%   The Simulink Function 'acadosSolve' (Subsystem2) is called by name.
%   Its arguments, in this order, feed the S-function inputs:
%     x0     (9)   -> lbx_0 and ubx_0      initial state equality = x0bar
%     ptraj  (272) -> parameter_traj       p of nodes 0..15, 17 each
%     yref0  (7)   -> y_ref_0              reference of node 0
%     yref   (98)  -> y_ref                references of nodes 1..14
%     yrefe  (5)   -> y_ref_e              reference of node 15
%     xinit  (144) -> x_init               state initial guess (9 x 16)
%     uinit  (30)  -> u_init               input initial guess (2 x 15) = 0
%     piinit (135) -> pi_init              dynamics multipliers (9 x 15) = 0
%   Returns u0 = first optimal steering-rate pair [rad/s], acados status,
%   CPU time [s] and number of SQP iterations. Uopt holds u0 in column 1
%   only (the S-function returns just the first input).
Nac = 15;  np = 17;

% Heading reference on the same 2*pi branch as the initial state
% (otherwise a 2*pi offset would look like a huge heading error).
psiRef = unwrap(reference(3,:));
reference(3,:) = psiRef + 2*pi*round((x0bar(3) - psiRef(1))/(2*pi));

% Parameters of nodes 0..15: [aDes; A(:); b; epsilon]. Each face normal
% (row of A) is scaled to unit length, b by the same factor, so that
% A*corner - b is a distance in metres. epsilon (corner-motion
% allowance) = 0.
ptraj = zeros(np*(Nac+1), 1);
for k = 1:Nac+1
    Ak = Acorr(:,:,k);  bk = bcorr(:,k);
    nk = sqrt(sum(Ak.^2, 2));
    ptraj((k-1)*np + (1:np)) = [aDes(k); reshape(Ak./[nk nk], [], 1); bk./nk; zeros(4,1)];
end

% References: node 0 (7 = 5 tracked states + 2 zero rates),
% nodes 1..14 (7 x 14, node after node), node 15 (5, no input terms).
yref0 = [reference(:,1); 0; 0];
yref  = reshape([reference(:,2:Nac); zeros(2, Nac-1)], [], 1);
yrefe = reference(:, Nac+1);

% Initial guess (same as Stage I): roll-out states with column 1 = x0bar,
% zero rates, zero multipliers.
xInit = xGuess;  xInit(:,1) = x0bar(:);
[u0, st, tCpu, nIt] = acadosSolve(x0bar(:), ptraj, yref0, yref, yrefe, ...
    xInit(:), zeros(2*Nac,1), zeros(9*Nac,1));

solverStatus = double(st);  solveTime = double(tCpu);  sqpIter = double(nIt);
Uopt = zeros(2, Nac);  Uopt(:,1) = u0;
end


%--------------------------------------------------------------------------
function [Acorr, bcorr] = buildCorridors(x0bar, reference, P, M)
%BUILDCORRIDORS  Obstacle corridor for every acados node, from the costmap.
%   Each corridor is a rectangle aligned with the vehicle (4 half-planes
%   A*q <= b): the expanded footprint, grown towards front, back, left and
%   right until an occupied or unknown cell is reached (at most gMax).
%     node 0     : around the predicted start pose x0bar (contains the car)
%     nodes 1..15: around the reference pose of the node (planned path is
%                  collision-free with the same 0.5 m margin)
%   Acorr: 4 x 2 x 16 normals, bcorr: 4 x 16 offsets (rows: front, back,
%   left, right). The OCP keeps the 4 car corners inside (soft constraint).

Nac = 15;

Acorr = zeros(4, 2, Nac+1);
bcorr = zeros(4, Nac+1);

for k = 1:Nac+1
    if k == 1
        Xk = x0bar(1);  Yk = x0bar(2);  psik = x0bar(3);
    else
        Xk = reference(1,k);  Yk = reference(2,k);  psik = reference(3,k);
    end
    [Ak, bk] = corridorAtPose(Xk, Yk, psik, P, M);
    Acorr(:,:,k) = Ak;
    bcorr(:,k)   = bk;
end
end

%--------------------------------------------------------------------------
function [A, b] = corridorAtPose(X, Y, psi, P, M)
%CORRIDORATPOSE  Largest vehicle-aligned free rectangle around the footprint.
%   Footprint in vehicle coordinates (origin at rear axle):
%     l in [footprintBack, footprintFront], w in [-halfWidth, +halfWidth]
%   The rectangle is grown by gF, gB, gL, gR >= 0 (at most gMax each):
%     pass 1: front and back, looking only at cells in the lateral band of
%             the footprint;
%     pass 2: left and right, looking at cells in the longitudinal band of
%             the rectangle grown in pass 1 (this covers the corners).
%   Cells are squares; cp is their half-size projected on a vehicle axis,
%   so a cell is "beyond" a face only if it does not touch it.
%   Cells overlapping the footprint itself are ignored (they would be a
%   collision already).

gMax = 1.0;                            % maximum growth per side [m]

c = cos(psi);
s = sin(psi);

front0 = P.footprintFront;             % +2.71 m
back0  = P.footprintBack;              % -0.71 m
half0  = P.footprintHalfWidth;         %  1.328 m

% Half size of one costmap cell measured along the vehicle axes.
cp = M.cellHalf*(abs(c) + abs(s));

% Costmap cells that can matter: world box around footprint + gMax
% (plus one cell of margin), clipped to the map.
lMid  = 0.5*(front0 + back0);
halfL = 0.5*(front0 - back0) + gMax;
halfW = half0 + gMax;
cx = X + c*lMid;
cy = Y + s*lMid;
projX = halfL*abs(c) + halfW*abs(s) + 2*M.cellHalf;
projY = halfL*abs(s) + halfW*abs(c) + 2*M.cellHalf;

ix0 = max(0,          ceil((cx - projX - M.originX)/M.res));
ix1 = min(M.width-1,  floor((cx + projX - M.originX)/M.res));
iy0 = max(0,          ceil((cy - projY - M.originY)/M.res));
iy1 = min(M.height-1, floor((cy + projY - M.originY)/M.res));

% ---- Pass 1: grow front and back (lateral band = footprint width) ----
gF = gMax;
gB = gMax;
for iy = iy0:iy1
    for ix = ix0:ix1
        v = M.grid(iy+1, ix+1);
        if v >= 1.0 || v < 0.0                     % occupied or unknown
            dx = M.originX + ix*M.res - X;
            dy = M.originY + iy*M.res - Y;
            l  =  c*dx + s*dy;                     % along the vehicle
            w  = -s*dx + c*dy;                     % to the left
            if abs(w) < half0 + cp
                if l - cp >= front0
                    gF = min(gF, l - cp - front0);
                elseif l + cp <= back0
                    gB = min(gB, back0 - (l + cp));
                end
            end
        end
    end
end

% ---- Pass 2: grow left and right (longitudinal band = grown length) ----
gL = gMax;
gR = gMax;
for iy = iy0:iy1
    for ix = ix0:ix1
        v = M.grid(iy+1, ix+1);
        if v >= 1.0 || v < 0.0
            dx = M.originX + ix*M.res - X;
            dy = M.originY + iy*M.res - Y;
            l  =  c*dx + s*dy;
            w  = -s*dx + c*dy;
            if (l + cp > back0 - gB) && (l - cp < front0 + gF)
                if w - cp >= half0
                    gL = min(gL, w - cp - half0);
                elseif w + cp <= -half0
                    gR = min(gR, -half0 - (w + cp));
                end
            end
        end
    end
end

% ---- Half-planes A*q <= b (unit normals: front, back, left, right) ----
% pl, pw = rear-axle position projected on the vehicle axes.
pl =  c*X + s*Y;                       % pose projected on the vehicle axes
pw = -s*X + c*Y;

A = [ c,  s;
     -c, -s;
     -s,  c;
      s, -c];

b = [ pl + front0 + gF;
     -(pl + back0 - gB);
      pw + half0 + gL;
     -(pw - half0 - gR)];
end
